simulink model "AMDSB_sincrono"  (Simulink 7.7)
settings: Solver=ode45  StartTime=0.0  StopTime=10.0  MaxStep=1e-2  RelTol=1e-3
values from neighbouring files (symbols this model uses):
  Den = [1 1]    [AMDSB_demodulador_main.m]    (also in AMDSB_nao_linear_main.m; AMDSB_sincrono_main.m)
  Num = 1    [AMDSB_demodulador_main.m]    (also in AMDSB_nao_linear_main.m; AMDSB_sincrono_main.m)
settings Model: Creator=vparro  LastModifiedBy=vanderleiparro
settings DebuggingCC: StrictBusMsg=Warning

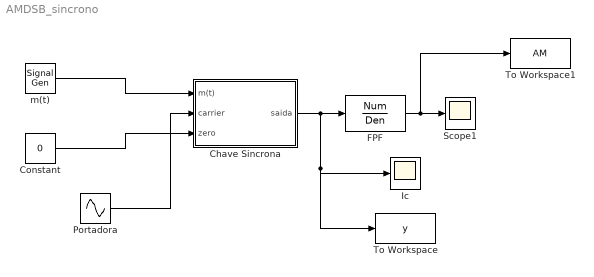
== system AMDSB_sincrono ==
  Chave Sincrona : Subsystem
  Constant : Constant  Value=0
  FPF : TransferFcn  Numerator=Num  Denominator=Den
  Ic : Scope
  Portadora : Sin  Frequency=20*pi  SampleTime=0
  Scope1 : Scope
  To Workspace : ToWorkspace  VariableName=y  SampleTime=-1  SaveFormat=Array
  To Workspace1 : ToWorkspace  VariableName=AM  SampleTime=-1  SaveFormat=Array
  m(t) : SignalGenerator  Units=rad/sec
  wires:
  FPF/1 -> Scope1/1, To Workspace1/1
  m(t)/1 -> Chave Sincrona/1(m(t))
  Constant/1 -> Chave Sincrona/3(zero)
  Portadora/1 -> Chave Sincrona/2(carrier)
  Chave Sincrona/1(saida) -> FPF/1, Ic/1, To Workspace/1

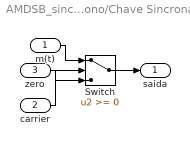
== system AMDSB_sincrono/Chave Sincrona ==
  m(t) : Inport
  carrier : Inport  Port=2
  zero : Inport  Port=3
  Switch : Switch
  saida : Outport
  wires:
  m(t)/1 -> Switch/1
  carrier/1 -> Switch/2
  Switch/1 -> saida/1
  zero/1 -> Switch/3
